simulink model "Es3_stateflow"  (R2025b)
settings: Solver=VariableStepAuto  StartTime=0.0  StopTime=10.0  RelTol=1e-3
settings Model: Creator=fsisa  LastModifiedBy=fsisa

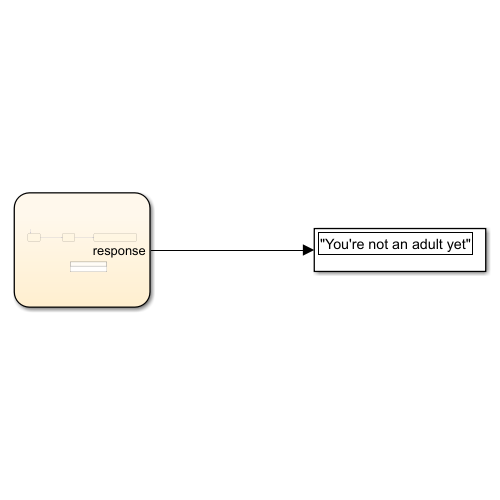
[thumbnail: Simulink's stored preview of the top-level diagram]
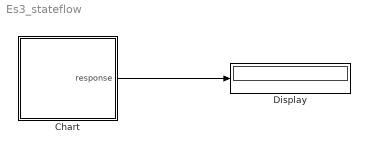
== system Es3_stateflow ==
  Chart : Stateflow chart  TreatAsAtomicUnit=on
  Display : Display
  wires:
  Chart/1(response) -> Display/1

== stateflow chart Es3_stateflow/Chart ==
  state Response
    response = CheckIfAdult(age)
  state Birth
    entry:
    age=0;
  state Growth
    during:
    age = age + 1;
  (default) -> Birth
  Growth -> Response : after(3,tick)
  Birth -> Growth : {age=age+1;}
  data: current_age function_input; response_check function_output; response output; age local
  function response_check = CheckIfAdult(current_age):
    | function response_check = CheckIfAdult(current_age)
    | 
    | if current_age >= 18
    |     response_check = "You're an adult now";
    | else
    |     response_check = "You're not an adult yet";
    | end
